simulink model "easy_ikSolver"  (R2025a)
settings: Solver=VariableStepAuto  StartTime=0.0  StopTime=10.0  RelTol=1e-3
values from neighbouring files (symbols this model uses):
  initialGuess = [0 0 0 0 0 0 0 0 0 0 0 0]    [robotInitialGuess.mat]
libraries: visiontextngfix x1, robotmaniplib x1
settings Model: Creator=matte  LastModifiedBy=matte

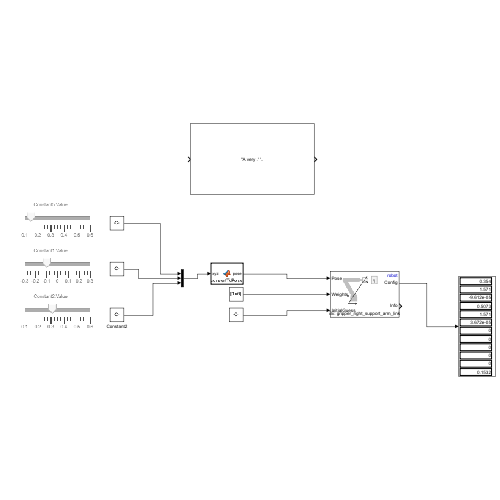
[thumbnail: Simulink's stored preview of the top-level diagram]
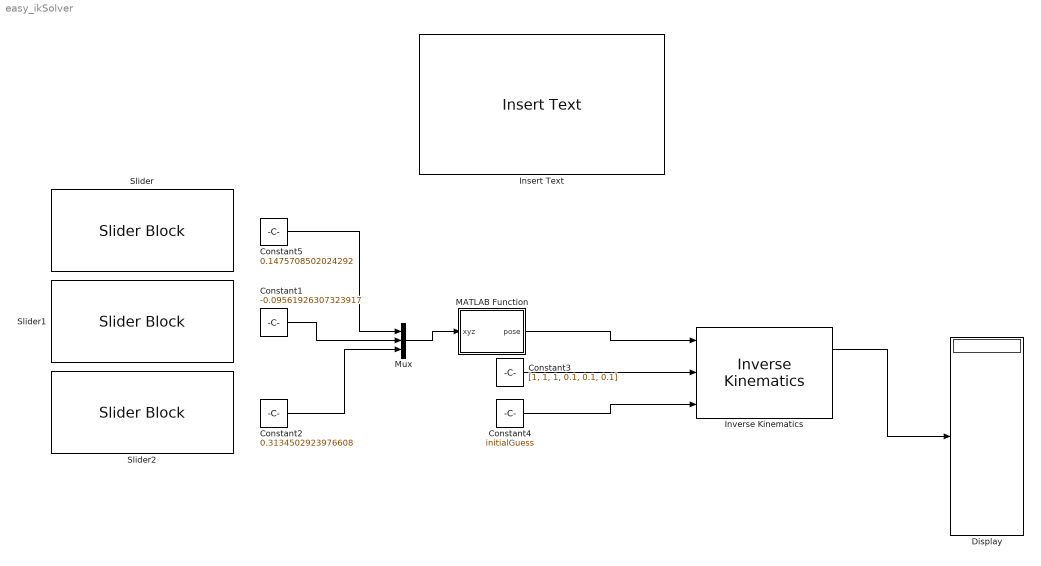
== system easy_ikSolver ==
  Constant1 : Constant  Value=-0.09561926307323917
  Constant2 : Constant  Value=0.3134502923976608
  Constant3 : Constant  Value=[1, 1, 1, 0.1, 0.1, 0.1]
  Constant4 : Constant  Value=initialGuess
  Constant5 : Constant  Value=0.1475708502024292
  Display : Display
  Insert Text : visiontextngfix/Insert Text  inputType=Obsolete  theText="\"A very primitive IK solver algorithm in Simulink\""  getTextLocFrom=Specify via dialog  textLoc=[1 1]  getTextColorFrom=Specify via dialog  textColor=[0 0 0]  getTextIntensityFrom=Specify via dialog  textIntensity=0  getTextOpacityFrom=Specify via dialog  textOpacity=1.0  dummyVar2=0  dummyVar3=0  dummyVar4=0  imagePorts=One multidimensional signal  isInputTransposed=off  fontFace=LucidaSansRegular  dummyVar1=0  blockFontSize=12  antiAliased=on
  Inverse Kinematics : robotmaniplib/Inverse Kinematics  RigidBodyTree=robot  EndEffector=gripper_right_support_arm_link  ShowInfo=on  SolverName=BFGS Gradient Projection  EnforceJointLimits=on  MaxIterations=1500  MaxTime=10  GradientTolerance=1e-7  SolutionTolerance=1e-6  StepTolerance=1e-14  ConstraintTolerance=1e-6  ErrorChangeTolerance=1e-12  UseErrorDamping=on  DampingBias=0.0025  SimulateUsing=Interpreted execution
  MATLAB Function : MATLAB Function  TreatAsAtomicUnit=on
  Mux : Mux  Inputs=3
  Slider : SliderBlock  ScaleMin=0.1  ScaleMax=0.6
  Slider1 : SliderBlock  ScaleMin=-0.3  ScaleMax=0.3
  Slider2 : SliderBlock  ScaleMin=0.1  ScaleMax=0.6
  wires:
  Constant5/1 -> Mux/1
  Constant3/1 -> Inverse Kinematics/2
  Inverse Kinematics/1 -> Display/1
  Constant4/1 -> Inverse Kinematics/3
  MATLAB Function/1(pose) -> Inverse Kinematics/1
  Mux/1 -> MATLAB Function/1(xyz)
  Constant2/1 -> Mux/3
  Constant1/1 -> Mux/2

== matlab function easy_ikSolver/MATLAB Function ==
  data: xyz input; pose output
function pose=convertToPose(xyz)
    x=xyz(1);
    y=xyz(2);
    z=xyz(3);

    pose=[
        1, 0, 0, x;
        0, 1, 0, y;
        0, 0, 1, z;
        0, 0, 0, 1;
    ];
    
end
